simulink model "W09_0_seam_demo"  (R2024b)
settings: Solver=FixedStepDiscrete  StartTime=0.0  StopTime=20  FixedStep=0.05  RelTol=1e-3
undefined symbols (not defined in the file or in its folder): DiscIntNeverNeededParam
settings Model: Creator=wkyou  LastModifiedBy=wkyou

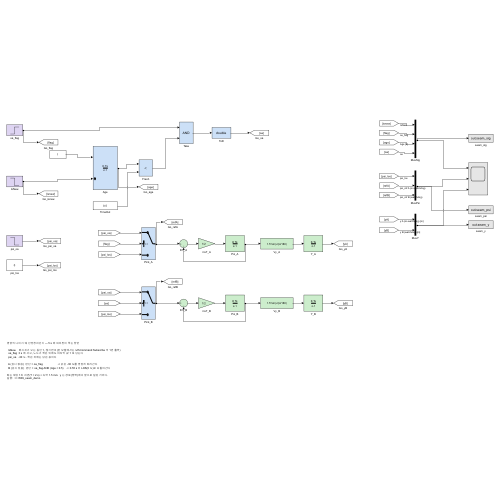
[thumbnail: Simulink's stored preview of the top-level diagram]
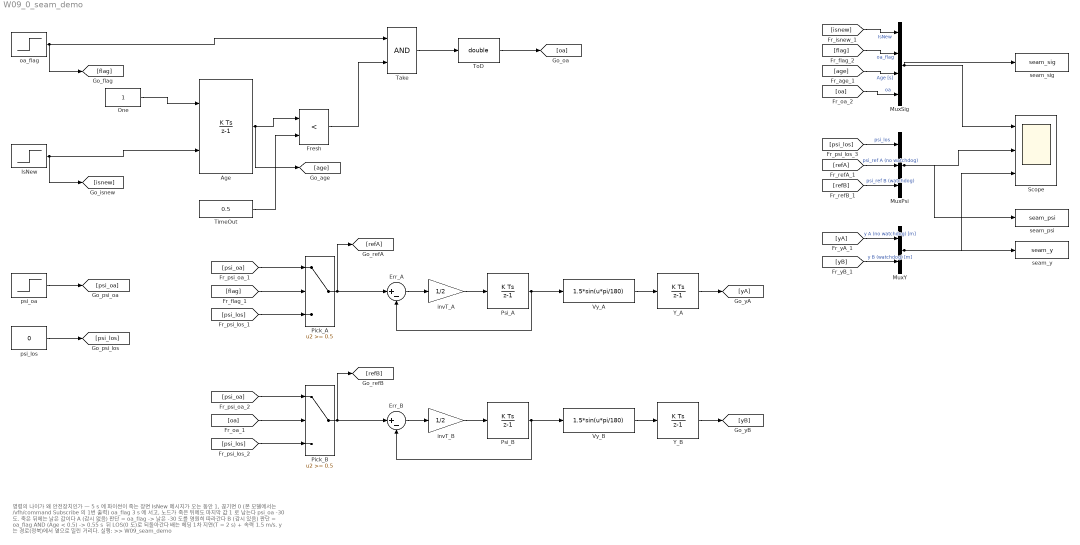
== system W09_0_seam_demo ==
  note: 명령의 나이가 왜 안전장치인가 — 5 s 에 파이썬이 죽는 장면
      |
      |   IsNew    메시지가 오는 동안 1, 끊기면 0 (본 모델에서는 /vfh/command Subscribe 의 1번 출력)
      |   oa_flag  3 s 에 서고, 노드가 죽은 뒤에도 마지막 값 1 로 남는다
      |   psi_oa   -30 도. 죽은 뒤에는 낡은 값이다
      |
      |   A (감시 없음)  판단 = oa_flag                    -> 낡은 -30 도를 영원히 따라간다
      |   B (감시 있음)  판단 = oa_flag AND (Age < 0.5)    -> 0.55 s 뒤 LOS(0 도)로 되돌아간다
      |
      | 배는 헤딩 1차 지연(T = 2 s) + 속력 1.5 m/s.  y 는 경로(정북)에서 옆으로 밀린 거리다.
      | 실행:  >> W09_seam_demo
  Age : DiscreteIntegrator  ExternalReset=level  SampleTime=0.05  ICPrevOutput=DiscIntNeverNeededParam  ICPrevScaledInput=DiscIntNeverNeededParam
  Err_A : Sum  Inputs=|+-
  Err_B : Sum  Inputs=|+-
  Fresh : RelationalOperator  Operator=<  OutDataTypeStr=boolean  RndMeth=Simplest  InputSameDT=off
  IsNew : Step  Time=5  Before=1  After=0  SampleTime=0.05
  MuxPsi : Mux  Inputs=3
  MuxSig : Mux
  MuxY : Mux  Inputs=2
  One : Constant  SampleTime=0.05
  Pick_A : Switch  Threshold=0.5  SaturateOnIntegerOverflow=off  InputSameDT=off
  Pick_B : Switch  Threshold=0.5  SaturateOnIntegerOverflow=off  InputSameDT=off
  Psi_A : DiscreteIntegrator  SampleTime=0.05  ICPrevOutput=DiscIntNeverNeededParam  ICPrevScaledInput=DiscIntNeverNeededParam
  Psi_B : DiscreteIntegrator  SampleTime=0.05  ICPrevOutput=DiscIntNeverNeededParam  ICPrevScaledInput=DiscIntNeverNeededParam
  Scope : Scope  NumInputPorts=3
  Take : Logic  AllPortsSameDT=off  OutDataTypeStr=boolean
  TimeOut : Constant  Value=0.5  SampleTime=0.05
  ToD : DataTypeConversion  OutDataTypeStr=double  SaturateOnIntegerOverflow=off  RndMeth=Floor
  Vy_A : Fcn  Expr=1.5*sin(u*pi/180)
  Vy_B : Fcn  Expr=1.5*sin(u*pi/180)
  Y_A : DiscreteIntegrator  SampleTime=0.05  ICPrevOutput=DiscIntNeverNeededParam  ICPrevScaledInput=DiscIntNeverNeededParam
  Y_B : DiscreteIntegrator  SampleTime=0.05  ICPrevOutput=DiscIntNeverNeededParam  ICPrevScaledInput=DiscIntNeverNeededParam
  invT_A : Gain  Gain=1/2
  invT_B : Gain  Gain=1/2
  oa_flag : Step  Time=3  SampleTime=0.05
  psi_los : Constant  Value=0  SampleTime=0.05
  psi_oa : Step  Time=3  After=-30  SampleTime=0.05
  seam_psi : ToWorkspace  VariableName=seam_psi  SaveFormat=Timeseries  SampleTime=-1
  seam_sig : ToWorkspace  VariableName=seam_sig  SaveFormat=Timeseries  SampleTime=-1
  seam_y : ToWorkspace  VariableName=seam_y  SaveFormat=Timeseries  SampleTime=-1
  wires:
  oa_flag/1 -> Take/1, [flag]
  One/1 -> Age/1
  IsNew/1 -> Age/2, [isnew]
  Age/1 -> Fresh/1, [age]
  TimeOut/1 -> Fresh/2
  Fresh/1 -> Take/2
  Take/1 -> ToD/1
  ToD/1 -> [oa]
  psi_oa/1 -> [psi_oa]
  psi_los/1 -> [psi_los]
  [psi_oa] -> Pick_A/1
  [flag] -> Pick_A/2
  [psi_los] -> Pick_A/3
  Pick_A/1 -> Err_A/1, [refA]
  Err_A/1 -> invT_A/1
  invT_A/1 -> Psi_A/1
  Psi_A/1 -> Vy_A/1, Err_A/2
  Vy_A/1 -> Y_A/1
  Y_A/1 -> [yA]
  [psi_oa] -> Pick_B/1
  [oa] -> Pick_B/2
  [psi_los] -> Pick_B/3
  Pick_B/1 -> Err_B/1, [refB]
  Err_B/1 -> invT_B/1
  invT_B/1 -> Psi_B/1
  Psi_B/1 -> Vy_B/1, Err_B/2
  Vy_B/1 -> Y_B/1
  Y_B/1 -> [yB]
  [isnew] -> MuxSig/1  "IsNew"
  [flag] -> MuxSig/2  "oa_flag"
  [age] -> MuxSig/3  "Age [s]"
  [oa] -> MuxSig/4  "oa"
  [psi_los] -> MuxPsi/1  "psi_los"
  [refA] -> MuxPsi/2  "psi_ref A (no watchdog)"
  [refB] -> MuxPsi/3  "psi_ref B (watchdog)"
  [yA] -> MuxY/1  "y A (no watchdog) [m]"
  [yB] -> MuxY/2  "y B (watchdog) [m]"
  MuxSig/1 -> Scope/1, seam_sig/1
  MuxPsi/1 -> Scope/2, seam_psi/1
  MuxY/1 -> Scope/3, seam_y/1
